simulink model "companion_io"  (R2026b)
settings: Solver=VariableStepAuto
undefined symbols (not defined in the file or in its folder): P, Ts
libraries: simulink x1
settings Model: Creator=aomar  LastModifiedBy=aomar

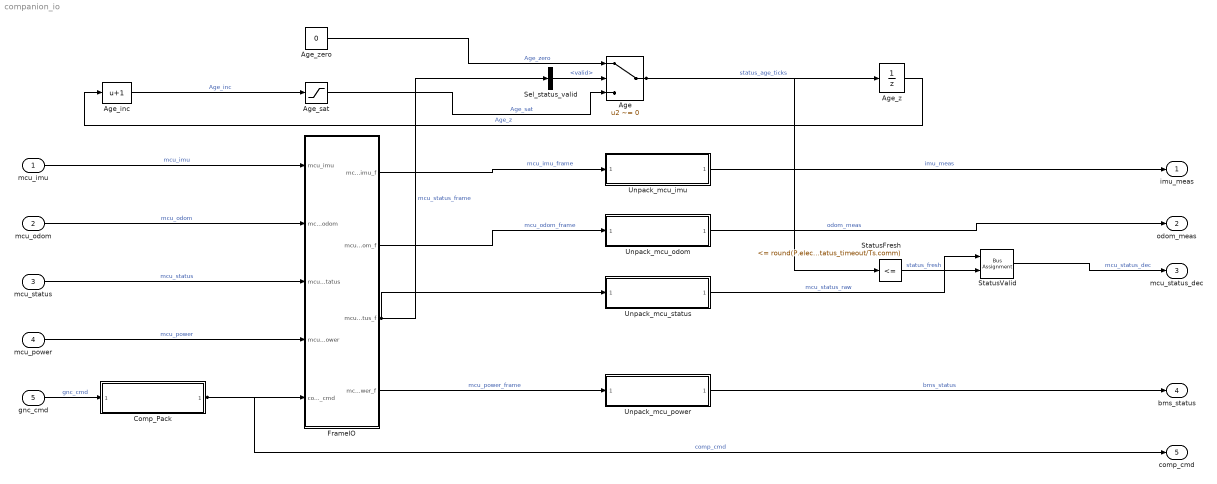
== system companion_io ==
  mcu_imu : Inport  OutDataTypeStr=Bus: Bus_CanFrame64  SampleTime=Ts.imu
  mcu_odom : Inport  Port=2  OutDataTypeStr=Bus: Bus_CanFrame64  SampleTime=Ts.ctrl
  mcu_status : Inport  Port=3  OutDataTypeStr=Bus: Bus_CanFrame64  SampleTime=Ts.comm
  mcu_power : Inport  Port=4  OutDataTypeStr=Bus: Bus_CanFrame64  SampleTime=Ts.hk
  gnc_cmd : Inport  Port=5  OutDataTypeStr=Bus: Bus_GncCmd  SampleTime=Ts.comm
  Age : Switch  Criteria=u2 ~= 0  SaturateOnIntegerOverflow=off  InputSameDT=off
  Age_inc : Bias  Bias=1  SaturateOnIntegerOverflow=off
  Age_sat : Saturate  UpperLimit=round(P.electronics.can.age_sat_s/Ts.comm)  LowerLimit=0
  Age_z : UnitDelay  InitialCondition=round(P.electronics.can.age_sat_s/Ts.comm)  SampleTime=Ts.comm
  Age_zero : Constant  Value=0  OutDataTypeStr=double  SampleTime=Ts.comm
  Comp_Pack : Subsystem  ReferencedSubsystem=can2_comp_cmd_pack
  FrameIO : Subsystem  Variant=on
  Sel_status_valid : BusSelector  OutputSignals=valid
  StatusFresh : simulink/Logic and Bit Operations/Compare To Constant  relop=<=  const=round(P.electronics.can.mcu_status_timeout/Ts.comm)  OutDataTypeStr=boolean
  StatusValid : BusAssignment  AssignedSignals=valid
  Unpack_mcu_imu : Subsystem  ReferencedSubsystem=can2_mcu_imu_unpack
  Unpack_mcu_odom : Subsystem  ReferencedSubsystem=can2_mcu_odom_unpack
  Unpack_mcu_power : Subsystem  ReferencedSubsystem=can2_mcu_power_unpack
  Unpack_mcu_status : Subsystem  ReferencedSubsystem=can2_mcu_status_unpack
  imu_meas : Outport  OutDataTypeStr=Bus: Bus_ImuMeas
  odom_meas : Outport  Port=2  OutDataTypeStr=Bus: Bus_OdomMeas
  mcu_status_dec : Outport  Port=3  OutDataTypeStr=Bus: Bus_McuStatus
  bms_status : Outport  Port=4  OutDataTypeStr=Bus: Bus_BmsStatus
  comp_cmd : Outport  Port=5  OutDataTypeStr=Bus: Bus_CanFrame64
  wires:
  mcu_imu/1 -> FrameIO/1(mcu_imu)  "mcu_imu"
  mcu_odom/1 -> FrameIO/2(mcu_odom)  "mcu_odom"
  mcu_status/1 -> FrameIO/3(mcu_status)  "mcu_status"
  mcu_power/1 -> FrameIO/4(mcu_power)  "mcu_power"
  gnc_cmd/1 -> Comp_Pack/1  "gnc_cmd"
  Age_inc/1 -> Age_sat/1  "Age_inc"
  Comp_Pack/1 -> comp_cmd/1, FrameIO/5(comp_cmd)  "comp_cmd"
  Age_zero/1 -> Age/1  "Age_zero"
  Age_sat/1 -> Age/3  "Age_sat"
  FrameIO/1(mcu_imu_f) -> Unpack_mcu_imu/1  "mcu_imu_frame"
  FrameIO/2(mcu_odom_f) -> Unpack_mcu_odom/1  "mcu_odom_frame"
  FrameIO/3(mcu_status_f) -> Sel_status_valid/1, Unpack_mcu_status/1  "mcu_status_frame"
  FrameIO/4(mcu_power_f) -> Unpack_mcu_power/1  "mcu_power_frame"
  Sel_status_valid/1 -> Age/2  "<valid>"
  Age/1 -> StatusFresh/1, Age_z/1  "status_age_ticks"
  Unpack_mcu_imu/1 -> imu_meas/1  "imu_meas"
  Unpack_mcu_odom/1 -> odom_meas/1  "odom_meas"
  Unpack_mcu_status/1 -> StatusValid/1  "mcu_status_raw"
  Unpack_mcu_power/1 -> bms_status/1  "bms_status"
  StatusFresh/1 -> StatusValid/2  "status_fresh"
  Age_z/1 -> Age_inc/1  "Age_z"
  StatusValid/1 -> mcu_status_dec/1  "mcu_status_dec"

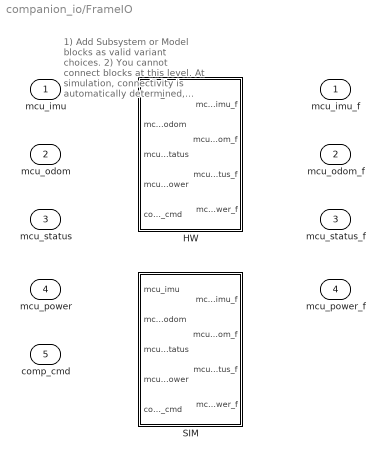
== system companion_io/FrameIO ==
  note: 1) Add Subsystem or Model blocks as valid variant choices.
      | 2) You cannot connect blocks at this level. At simulation, connectivity is automatically
      | determined, based on the active variant and port name matching.
  mcu_imu : Inport
  mcu_odom : Inport  Port=2
  mcu_status : Inport  Port=3
  mcu_power : Inport  Port=4
  comp_cmd : Inport  Port=5
  HW : Subsystem  VariantControl=VC_TARGET == 1
  SIM : Subsystem  VariantControl=VC_TARGET == 0
  mcu_imu_f : Outport
  mcu_odom_f : Outport  Port=2
  mcu_status_f : Outport  Port=3
  mcu_power_f : Outport  Port=4

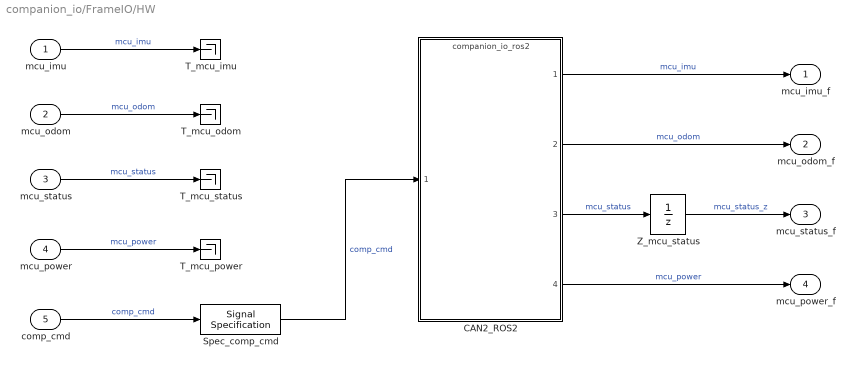
== system companion_io/FrameIO/HW ==
  mcu_imu : Inport
  mcu_odom : Inport  Port=2
  mcu_status : Inport  Port=3
  mcu_power : Inport  Port=4
  comp_cmd : Inport  Port=5
  CAN2_ROS2 : ModelReference  ModelNameDialog=companion_io_ros2  SimulationMode=Normal  ModelReferenceVersion=1.1
  Spec_comp_cmd : SignalSpecification  OutDataTypeStr=Bus: Bus_CanFrame64  SampleTime=Ts.comm  BusOutputAsStruct=on
  T_mcu_imu : Terminator
  T_mcu_odom : Terminator
  T_mcu_power : Terminator
  T_mcu_status : Terminator
  Z_mcu_status : UnitDelay  InitialCondition=P.ic.Bus_CanFrame64  SampleTime=Ts.gnc
  mcu_imu_f : Outport
  mcu_odom_f : Outport  Port=2
  mcu_status_f : Outport  Port=3
  mcu_power_f : Outport  Port=4
  wires:
  mcu_imu/1 -> T_mcu_imu/1  "mcu_imu"
  mcu_odom/1 -> T_mcu_odom/1  "mcu_odom"
  mcu_status/1 -> T_mcu_status/1  "mcu_status"
  mcu_power/1 -> T_mcu_power/1  "mcu_power"
  comp_cmd/1 -> Spec_comp_cmd/1  "comp_cmd"
  Spec_comp_cmd/1 -> CAN2_ROS2/1  "comp_cmd"
  CAN2_ROS2/1 -> mcu_imu_f/1  "mcu_imu"
  CAN2_ROS2/2 -> mcu_odom_f/1  "mcu_odom"
  CAN2_ROS2/3 -> Z_mcu_status/1  "mcu_status"
  CAN2_ROS2/4 -> mcu_power_f/1  "mcu_power"
  Z_mcu_status/1 -> mcu_status_f/1  "mcu_status_z"

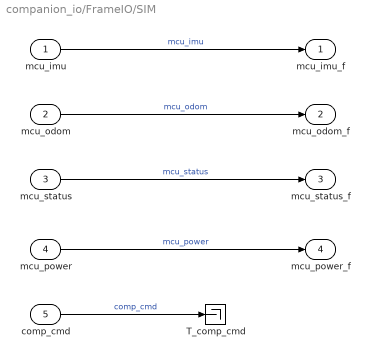
== system companion_io/FrameIO/SIM ==
  mcu_imu : Inport
  mcu_odom : Inport  Port=2
  mcu_status : Inport  Port=3
  mcu_power : Inport  Port=4
  comp_cmd : Inport  Port=5
  T_comp_cmd : Terminator
  mcu_imu_f : Outport
  mcu_odom_f : Outport  Port=2
  mcu_status_f : Outport  Port=3
  mcu_power_f : Outport  Port=4
  wires:
  mcu_imu/1 -> mcu_imu_f/1  "mcu_imu"
  mcu_odom/1 -> mcu_odom_f/1  "mcu_odom"
  mcu_status/1 -> mcu_status_f/1  "mcu_status"
  mcu_power/1 -> mcu_power_f/1  "mcu_power"
  comp_cmd/1 -> T_comp_cmd/1  "comp_cmd"
